simulink model "can_decoder"  (R2026a)
settings: configuration reference "AMCBLDC_Configuration" (kept outside this file)
undefined symbols (not defined in the file): CAN_ID_AMC, CAN_VOLT_REF_GAIN, CAN_VOLT_REF_SHIFT
settings Model: DataDictionary=amcbldc.sldd  Creator=upattacini  LastModifiedBy=rpumpo
settings ConfigSetRef: SourceName=AMCBLDC_Configuration

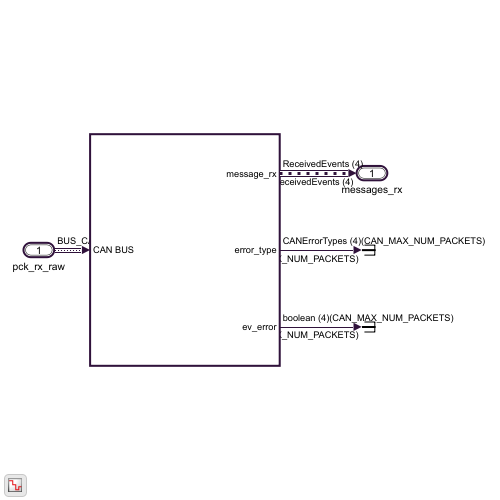
[thumbnail: Simulink's stored preview of the top-level diagram]
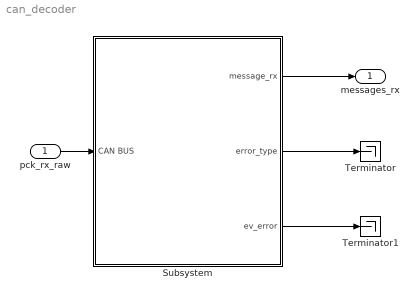
== system can_decoder ==
  pck_rx_raw : Inport  OutDataTypeStr=Bus: BUS_CAN_MULTIPLE  BusOutputAsStruct=on
  Subsystem : Subsystem
  Terminator : Terminator
  Terminator1 : Terminator
  messages_rx : Outport  OutDataTypeStr=Bus: ReceivedEvents  BusOutputAsStruct=on
  wires:
  pck_rx_raw/1 -> Subsystem/1(CAN BUS)
  Subsystem/1(message_rx) -> messages_rx/1
  Subsystem/2(error_type) -> Terminator/1
  Subsystem/3(ev_error) -> Terminator1/1

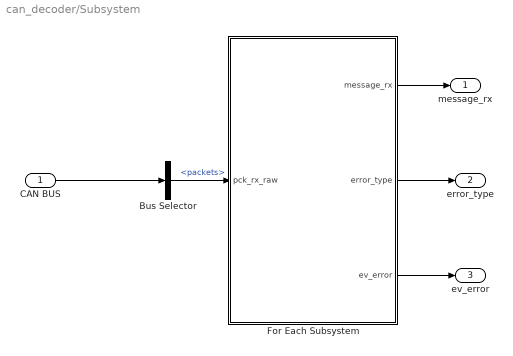
== system can_decoder/Subsystem ==
  CAN BUS : Inport
  Bus Selector : BusSelector  OutputSignals=packets
  For Each Subsystem : Subsystem  TreatAsAtomicUnit=on
  message_rx : Outport  PortDimensions=4
  error_type : Outport  Port=2
  ev_error : Outport  Port=3
  wires:
  Bus Selector/1 -> For Each Subsystem/1(pck_rx_raw)  "<packets>"
  CAN BUS/1 -> Bus Selector/1
  For Each Subsystem/3(ev_error) -> ev_error/1
  For Each Subsystem/1(message_rx) -> message_rx/1
  For Each Subsystem/2(error_type) -> error_type/1

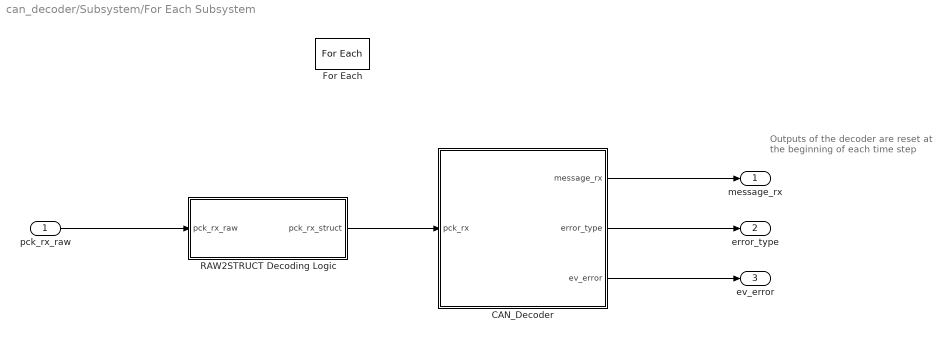
== system can_decoder/Subsystem/For Each Subsystem ==
  note: Outputs of the decoder are reset at
      | the beginning of each time step
  pck_rx_raw : Inport  Partition=on  PartitionDimension=1  PartitionWidth=1  PartitionOffset=0
  CAN_Decoder : Subsystem  TreatAsAtomicUnit=on
  For Each : ForEach  DisableCoverage=on  SpecifiedNumIters=MAX_EVENTS_PER_TICK
  RAW2STRUCT Decoding Logic : MATLAB Function  TreatAsAtomicUnit=on
  message_rx : Outport  OutDataTypeStr=Bus: ReceivedEvents  ConcatenationDimension=1
  error_type : Outport  Port=2  ConcatenationDimension=1
  ev_error : Outport  Port=3  ConcatenationDimension=1
  wires:
  CAN_Decoder/3(ev_error) -> ev_error/1
  RAW2STRUCT Decoding Logic/1(pck_rx_struct) -> CAN_Decoder/1(pck_rx)
  CAN_Decoder/1(message_rx) -> message_rx/1
  pck_rx_raw/1 -> RAW2STRUCT Decoding Logic/1(pck_rx_raw)
  CAN_Decoder/2(error_type) -> error_type/1

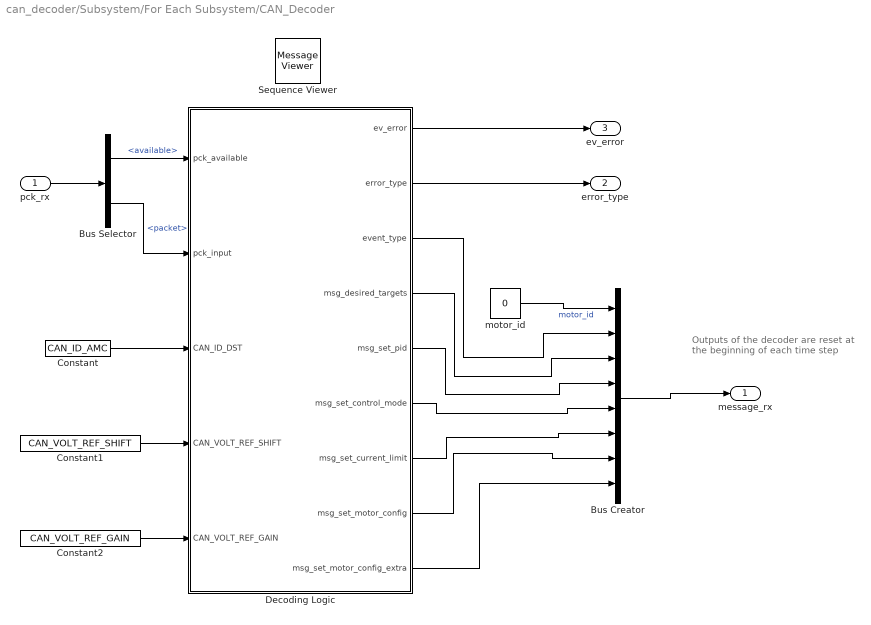
== system can_decoder/Subsystem/For Each Subsystem/CAN_Decoder ==
  note: Outputs of the decoder are reset at
      | the beginning of each time step
  pck_rx : Inport  OutDataTypeStr=Bus: BUS_CAN_RX
  Bus Creator : BusCreator  Inputs=8  OutDataTypeStr=Bus: ReceivedEvents  NonVirtualBus=on
      settings: InheritFromInputs=off
  Bus Selector : BusSelector  OutputSignals=available,packet
  Constant : Constant  Value=CAN_ID_AMC  OutDataTypeStr=uint8
  Constant1 : Constant  Value=CAN_VOLT_REF_SHIFT  OutDataTypeStr=uint8
  Constant2 : Constant  Value=CAN_VOLT_REF_GAIN  OutDataTypeStr=single
  Decoding Logic : Stateflow chart  TreatAsAtomicUnit=on
      settings: PortSchema="{\"entries\":[{\"content\":{\"sides\":[{\"content\":{\"connectorIds\":[\"In1\",\"In2\",\"In3\",\"In4\",\"In5\"]},\"type\":\"ConnectorPlacement.EquallySpacedRectSide\",\"uuid\":\"bb5ffdcb-390f-4d7b-9f99-b75bae8a05ad\"},{\"content\":{\"connectorIds\":[\"Out9\",\"Out6\",\"Out7\",\"Out3\",\"Out4\",\"Out1\",\"Out2\",\"Out5\",\"Out8\"],\"side\":\"RIGHT\"},\"type\":\"ConnectorPlacement.EquallySpacedRectSide\",\"uuid\":\"3ba90815-a3e4-4cd4-b64a-5c95e1f5d631\"},{\"content\":{\"side\":\"TOP\"},\"type\":\"ConnectorPlacement.EquallySpacedRectSide\",\"uuid\":\"c9c9b262-1031-4ca9-8b93-619604387376\"}]},\"type\":\"ConnectorPlacement.EquallySpacedConnector\",\"uuid\":\"025015ea-955c-40a8-a93e-b34368e10f0a\"}],\"packageUris\":[\"http://schema.mathworks.com/mf0/Connector/R2020b\"],\"version\":\"1.0\"}"
  Sequence Viewer : MessageViewer
  motor_id : Constant  Value=0  OutDataTypeStr=uint8
  message_rx : Outport  OutDataTypeStr=Bus: ReceivedEvents
  error_type : Outport  Port=2
  ev_error : Outport  Port=3
  wires:
  Constant/1 -> Decoding Logic/3(CAN_ID_DST)
  pck_rx/1 -> Bus Selector/1
  Bus Selector/1 -> Decoding Logic/1(pck_available)  "<available>"
  Bus Selector/2 -> Decoding Logic/2(pck_input)  "<packet>"
  Constant1/1 -> Decoding Logic/4(CAN_VOLT_REF_SHIFT)
  Constant2/1 -> Decoding Logic/5(CAN_VOLT_REF_GAIN)
  Decoding Logic/9(ev_error) -> ev_error/1
  Decoding Logic/6(error_type) -> error_type/1
  Bus Creator/1 -> message_rx/1
  Decoding Logic/7(event_type) -> Bus Creator/2
  Decoding Logic/3(msg_desired_targets) -> Bus Creator/3
  Decoding Logic/4(msg_set_pid) -> Bus Creator/4
  Decoding Logic/1(msg_set_control_mode) -> Bus Creator/5
  Decoding Logic/2(msg_set_current_limit) -> Bus Creator/6
  Decoding Logic/5(msg_set_motor_config) -> Bus Creator/7
  motor_id/1 -> Bus Creator/1  "motor_id"
  Decoding Logic/8(msg_set_motor_config_extra) -> Bus Creator/8

== matlab function can_decoder/Subsystem/For Each Subsystem/RAW2STRUCT Decoding Logic ==
  data: pck_rx_raw input Bus: BUS_CAN; pck_rx_struct output Bus: BUS_CAN_RX
function pck_rx_struct = raw2struct(pck_rx_raw)

pck_rx_struct.available = pck_rx_raw.available;

% ID
pck_rx_struct.packet.ID.CLS = CANClassTypes(bitshift(bitand(pck_rx_raw.packet.ID, 0x0700), -8));
pck_rx_struct.packet.ID.SRC = uint8(bitshift(bitand(pck_rx_raw.packet.ID, 0x0f0), -4));
pck_rx_struct.packet.ID.DST_TYP = uint8(bitand(pck_rx_raw.packet.ID, 0x00f));

% PAYLOAD
pck_rx_struct.packet.PAYLOAD.LEN = max([0, min([8, pck_rx_raw.length])]);
pck_rx_struct.packet.PAYLOAD.CMD.M = (bitand(pck_rx_raw.packet.PAYLOAD(1), 0x80) ~= 0);
pck_rx_struct.packet.PAYLOAD.CMD.OPC = bitand(pck_rx_raw.packet.PAYLOAD(1), 0x7f);
% We get both the polling and the streaming packtes covered
pck_rx_struct.packet.PAYLOAD.ARG = pck_rx_raw.packet.PAYLOAD;

== stateflow chart can_decoder/Subsystem/For Each Subsystem/CAN_Decoder/Decoding Logic ==
  settings: initializeOutput=1  description=This state chart is responsible for decoding incoming CAN packets.
  state ErrorHandler [parallel]
    settings: executionOrder=2
    state Home
      entry:
      cmd_processed = 0;
      exit:
      ev_async = false;
    state Event_Error
      entry:
      ev_async = true;
    (default) -> ErrorHandler.Home
    (junction 111) -> ErrorHandler.Home [order 2] : {error_type = CANErrorTypes.No_Error;}
    (junction 111) -> ErrorHandler.Home [order 1] : [cmd_processed > 1]
        | {error_type = CANErrorTypes.Packet_MultiFunctionsDetected;
        | send(ev_error);}
    ErrorHandler.Home -> ErrorHandler.Home [order 4] : [ev_async]
    (junction 109) -> ErrorHandler.Home [order 1] : [pck_available && (cmd_processed == 0)]
        | {error_type = CANErrorTypes.Packet_Unrecognized;
        | send(ev_error);}
    Event_Error -> ErrorHandler.Home
    ErrorHandler.Home -> (junction 109) [order 5]
    ErrorHandler.Home -> Event_Error [order 1] : ev_error_pck_not4us
        | {error_type = CANErrorTypes.Packet_Not4Us;
        | send(ev_error);}
    ErrorHandler.Home -> Event_Error [order 2] : ev_error_pck_malformed
        | {error_type = CANErrorTypes.Packet_Malformed;
        | send(ev_error);}
    ErrorHandler.Home -> Event_Error [order 3] : ev_error_mode_unrecognized
        | {error_type = CANErrorTypes.Mode_Unrecognized;
        | send(ev_error);}
    (junction 109) -> (junction 111) [order 2]
  state CANParser [parallel]
    settings: executionOrder=1
    state Home
    state SetCommand [function]
      state r = isPayloadValid(expected_size) [function]
        (default) -> (junction 402) : {r = true;}
        (junction 402) -> (junction 503) [order 1] : [pck_input.ID.DST_TYP != CAN_ID_DST]{send(ev_error_pck_not4us, ErrorHandler); r = false;}
        (junction 402) -> (junction 505) [order 2] : [pck_input.PAYLOAD.LEN < 1]{send(ev_error_pck_malformed, ErrorHandler); r = false;}
        (junction 402) -> (junction 507) [order 3] : [pck_input.PAYLOAD.LEN <  expected_size]
            | {send(ev_error_pck_malformed, ErrorHandler);; r = false;}
      state SetControlMode [function]
        (default) -> (junction 510)
        (junction 510) -> (junction 339) [order 2] : {mc_mode =  pck_input.PAYLOAD.ARG[1];}
        (junction 339) -> (junction 406) [order 2] : {% msg_set_control_mode.motor = pck_input.PAYLOAD.CMD.M;
            | msg_set_control_mode = convertMode(mc_mode);
            | cmd_processed++;
            | event_type = EventTypes.SetControlMode;}
        (junction 339) -> (junction 408) [order 1] : [!is_controlmode_recognized(mc_mode)]
            | {send(ev_error_mode_unrecognized, ErrorHandler);}
        (junction 510) -> (junction 523) [order 1] : [!isPayloadValid(2)]
      state SetCurrentLimits [function]
        (default) -> (junction 381)
        (junction 381) -> (junction 527) [order 1] : [!isPayloadValid(8)]
        (junction 381) -> (junction 382) [order 2] : {% msg_set_current_limit.motor = pck_input.PAYLOAD.CMD.M;
            | msg_set_current_limit.nominal = single(0.001)*single(merge_2bytes_signed(pck_input.PAYLOAD.ARG[2], pck_input.PAYLOAD.ARG[3]));
            | msg_set_current_limit.peak = single(0.001)*single(merge_2bytes_unsigned(pck_input.PAYLOAD.ARG[4], pck_input.PAYLOAD.ARG[5]));
            | msg_set_current_limit.overload = single(0.001)*single(merge_2bytes_unsigned(pck_input.PAYLOAD.ARG[6], pck_input.PAYLOAD.ARG[7]));
            | cmd_processed++;
            | event_type = EventTypes.SetLimit;}
      state SetMotorConfig [function]
        (default) -> (junction 397)
        (junction 397) -> (junction 530) [order 1] : [!isPayloadValid(8)]
        (junction 397) -> (junction 398) [order 2] : {msg_set_motor_config.has_quadrature_encoder = boolean(pck_input.PAYLOAD.ARG[1] & 0x01);
            | msg_set_motor_config.has_hall_sens = boolean(pck_input.PAYLOAD.ARG[1] & 0x02);
            | msg_set_motor_config.has_temperature_sens = boolean(pck_input.PAYLOAD.ARG[1] & 0x04);
            | msg_set_motor_config.use_index = boolean(pck_input.PAYLOAD.ARG[1] & 0x08);
            | msg_set_motor_config.has_speed_quadrature_encoder = boolean(pck_input.PAYLOAD.ARG[1] & 0x10);
            | msg_set_motor_config.enable_verbosity = boolean(pck_input.PAYLOAD.ARG[1] & 0x20);
            | msg_set_motor_config.rotor_encoder_resolution = merge_2bytes_signed(pck_input.PAYLOAD.ARG[2], pck_input.PAYLOAD.ARG[3]);
            | msg_set_motor_config.rotor_index_offset = merge_2bytes_signed(pck_input.PAYLOAD.ARG[4], pck_input.PAYLOAD.ARG[5]);
            | msg_set_motor_config.pole_pairs = pck_input.PAYLOAD.ARG[6] / 2;
            | msg_set_motor_config.encoder_tolerance = pck_input.PAYLOAD.ARG[7];
            | cmd_processed++;
            | event_type = EventTypes.SetMotorConfig;}
      state SetCurrentPID [function]
        (default) -> (junction 386)
        (junction 386) -> (junction 387) [order 2] : {%msg_set_pid.motor = pck_input.PAYLOAD.CMD.M;
            | msg_set_pid.shift_factor = pck_input.PAYLOAD.ARG[7];
            | c = single(0x01 << (15 - msg_set_pid.shift_factor)) / single(32768);
            | msg_set_pid.P = c * single(merge_2bytes_signed(pck_input.PAYLOAD.ARG[1], pck_input.PAYLOAD.ARG[2]));
            | msg_set_pid.I = c * single(merge_2bytes_signed(pck_input.PAYLOAD.ARG[3], pck_input.PAYLOAD.ARG[4]));
            | msg_set_pid.D = c * single(merge_2bytes_signed(pck_input.PAYLOAD.ARG[5], pck_input.PAYLOAD.ARG[6]));
            | msg_set_pid.type = ControlModes.Current;
            | event_type = EventTypes.SetPid;
            | cmd_processed++;}
        (junction 386) -> (junction 532) [order 1] : [!isPayloadValid(8)]
      state SetVelocityPID [function]
        (default) -> (junction 391)
        (junction 391) -> (junction 392) [order 2] : {msg_set_pid.shift_factor = pck_input.PAYLOAD.ARG[7];
            | c = single(0x01 << (15 - msg_set_pid.shift_factor)) / single(32768);
            | msg_set_pid.P = c * single(merge_2bytes_signed(pck_input.PAYLOAD.ARG[1], pck_input.PAYLOAD.ARG[2]));
            | msg_set_pid.I = c * single(merge_2bytes_signed(pck_input.PAYLOAD.ARG[3], pck_input.PAYLOAD.ARG[4]));
            | msg_set_pid.D = c * single(merge_2bytes_signed(pck_input.PAYLOAD.ARG[5], pck_input.PAYLOAD.ARG[6]));
            | msg_set_pid.P *= single(0.001);
            | msg_set_pid.I *= single(0.001);
            | msg_set_pid.D *= single(0.001);
            | msg_set_pid.type = ControlModes.Velocity;
            | event_type = EventTypes.SetPid;
            | cmd_processed++;}
        (junction 391) -> (junction 534) [order 1] : [!isPayloadValid(8)]
      state SetPositionPID [function]
        (default) -> (junction 826)
        (junction 826) -> (junction 827) [order 2] : {msg_set_pid.shift_factor = pck_input.PAYLOAD.ARG[7];
            | c = single(0x01 << (15 - msg_set_pid.shift_factor)) / single(32768);
            | msg_set_pid.P = c * single(merge_2bytes_signed(pck_input.PAYLOAD.ARG[1], pck_input.PAYLOAD.ARG[2]));
            | msg_set_pid.I = c * single(merge_2bytes_signed(pck_input.PAYLOAD.ARG[3], pck_input.PAYLOAD.ARG[4]));
            | msg_set_pid.D = c * single(merge_2bytes_signed(pck_input.PAYLOAD.ARG[5], pck_input.PAYLOAD.ARG[6]));
            | msg_set_pid.type = ControlModes.Position;
            | event_type = EventTypes.SetPid;
            | cmd_processed++;}
        (junction 826) -> (junction 825) [order 1] : [!isPayloadValid(8)]
      state SetMotorParameter [function]
        (default) -> (junction 747)
        (junction 747) -> (junction 731) [order 2] : {p = pck_input.PAYLOAD.ARG[1];}
        (junction 731) -> (junction 722) [order 1] : [p == MCMotorParamsSet.Kbemf]
        (junction 722) -> (junction 715) : {msg_set_motor_config_extra.value = ...
            | merge_4bytes_single(pck_input.PAYLOAD.ARG);}
        (junction 747) -> (junction 809) [order 1] : [!isPayloadValid(8)]
        (junction 731) -> (junction 718) [order 2]
        (junction 715) -> (junction 714)
        (junction 718) -> (junction 719) [order 1] : [p == MCMotorParamsSet.hall]
        (junction 719) -> (junction 714) : {msg_set_motor_config_extra.value = ...
            | unpack_hall_config(pck_input.PAYLOAD.ARG);}
        (junction 718) -> (junction 717) [order 2]
        (junction 714) -> (junction 738)
        (junction 717) -> (junction 723) [order 1] : [p == MCMotorParamsSet.elect_vmax]
        (junction 723) -> (junction 738) : {msg_set_motor_config_extra.value = ...
            | merge_4bytes_single(pck_input.PAYLOAD.ARG);}
        (junction 717) -> (junction 740) [order 2]
        (junction 738) -> (junction 739)
        (junction 739) -> (junction 740) : {msg_set_motor_config_extra.key = p;}
        (junction 740) -> (junction 742) : {event_type = EventTypes.SetMotorParam;}
      state Set [function]
        (default) -> (junction 877)
        (junction 877) -> (junction 878) : [(pck_input.PAYLOAD.LEN == 8) && (CAN_ID_DST <= 4)]
            | {
            |  [msg_desired_targets.position,msg_desired_targets.velocity] = decode_pos_vel(pck_input.PAYLOAD.ARG);
            | cmd_processed++;
            | event_type = EventTypes.SetTarget;}
      (default) -> (junction 310)
      (junction 310) -> (junction 312) [order 1] : [pck_input.PAYLOAD.CMD.OPC == MCOPC.Set_Control_Mode]
          | {SetControlMode();}
      (junction 310) -> (junction 314) [order 2]
      (junction 312) -> (junction 316)
      (junction 314) -> (junction 316) [order 1] : [pck_input.PAYLOAD.CMD.OPC == MCOPC.Set_Current_Limit]
          | {SetCurrentLimits();}
      (junction 314) -> (junction 318) [order 2]
      (junction 316) -> (junction 321)
      (junction 318) -> (junction 321) [order 1] : [pck_input.PAYLOAD.CMD.OPC == MCOPC.Set_Motor_Config]
          | {SetMotorConfig();}
      (junction 318) -> (junction 324) [order 2]
      (junction 321) -> (junction 322)
      (junction 324) -> (junction 322) [order 1] : [pck_input.PAYLOAD.CMD.OPC == MCOPC.Set_Current_PID]
          | {SetCurrentPID();}
      (junction 324) -> (junction 328) [order 2]
      (junction 322) -> (junction 326)
      (junction 328) -> (junction 326) [order 1] : [pck_input.PAYLOAD.CMD.OPC == MCOPC.Set_Velocity_PID]
          | {SetVelocityPID();}
      (junction 326) -> (junction 819)
      (junction 328) -> (junction 821) [order 2]
      (junction 821) -> (junction 819) [order 1] : [pck_input.PAYLOAD.CMD.OPC == MCOPC.Set_Position_PID]
          | {SetPositionPID();}
      (junction 821) -> (junction 614) [order 2]
      (junction 819) -> (junction 618)
      (junction 614) -> (junction 618) [order 1] : [pck_input.PAYLOAD.CMD.OPC == MCOPC.Set_Parameter]
          | {SetMotorParameter();}
      (junction 618) -> (junction 576)
      (junction 614) -> (junction 334) [order 2]
      (junction 334) -> (junction 576) [order 1] : [pck_input.PAYLOAD.CMD.OPC == MCOPC.Set]
          | {Set();}
      (junction 334) -> (junction 831) [order 2]
      (junction 576) -> (junction 834)
      (junction 834) -> (junction 831)
      (junction 831) -> (junction 579)
    state SetStreaming [function]
      state SetTargets [function]
        (default) -> (junction 372)
        (junction 372) -> (junction 373) : [(pck_input.PAYLOAD.LEN == 8) && (CAN_ID_DST <= 4)]
            | {idx = 2*(CAN_ID_DST-1);
            | tmp_merged = merge_2bytes_signed(pck_input.PAYLOAD.ARG[idx], pck_input.PAYLOAD.ARG[idx+1]);
            | msg_desired_targets.current = single(0.001) * single(tmp_merged);
            | msg_desired_targets.voltage = single(tmp_merged >> CAN_VOLT_REF_SHIFT) / CAN_VOLT_REF_GAIN;
            | msg_desired_targets.velocity = single(1000) * single(tmp_merged) * CAN_ANGLE_ICUB2DEG;
            | cmd_processed++;
            | event_type = EventTypes.SetTarget;}
      (default) -> (junction 344)
      (junction 344) -> (junction 345) : [ (MCStreaming(pck_input.ID.DST_TYP) == MCStreaming.Desired_Targets)]
          | {SetTargets();}
    (default) -> CANParser.Home
    CANParser.Home -> (junction 535) : [pck_available]
    (junction 535) -> (junction 303) [order 1] : [(pck_input.ID.CLS == CANClassTypes.Motor_Control_Command)]
        | {SetCommand();}
    (junction 535) -> CANParser.Home [order 3]
    (junction 535) -> (junction 303) [order 2] : [(pck_input.ID.CLS == CANClassTypes.Motor_Control_Streaming)]
        | {SetStreaming();}
    (junction 303) -> CANParser.Home
  data: ev_async local boolean =false; expected_size function_input uint8; r function_output boolean; MCMode function_input Enum: MCControlModes; mode function_output Enum: ControlModes; mode function_input int32; ok function_output boolean; d function_input uint8 size=8; sw function_output single size=[2, 1]; hall_data function_output single size=[2, 1]; d function_input uint8 size=8; payload function_input uint8 size=[1,8]; target_pos function_output single; target_vel function_output single; hex function_input uint16; decimal_value function_output single; bl function_input uint16; bh function_input uint16; uw function_output uint16; bl function_input uint16; bh function_input uint16; sw function_output int16; pck_available input boolean; pck_input input Bus: BUS_CAN_PACKET_RX; CAN_ID_DST input uint8; msg_set_control_mode output Enum: ControlModes; msg_set_current_limit output Bus: SupervisorInputLimits; msg_desired_targets output Bus: Targets; msg_set_pid output Bus: PID; msg_set_motor_config output Bus: MotorConfigurationExternal; error_type output Enum: CANErrorTypes size=1 =CANErrorTypes.No_Error; cmd_processed local uint16 size=1 =0; CAN_VOLT_REF_SHIFT input uint8; CAN_VOLT_REF_GAIN input single; CAN_ANGLE_ICUB2DEG parameter; event_type output Enum: EventTypes =EventTypes.None; c local double; tmp_merged local double; idx local double; mc_mode local double; p local uint8; msg_set_motor_config_extra output Bus: MotorConfigurationExtSet
  data CAN_ID_DST settings: description=The ID of the receiver.
  data msg_set_control_mode settings: description=Contains the data to set the required control mode.
  data msg_set_current_limit settings: description=Contains the data to set the required current limit.
  data msg_desired_targets settings: description=Contains the data to set the required current limit.
  data msg_set_pid settings: description=Contains the data to set the required current limit.
  data msg_set_motor_config settings: description=Contains the data to set the required current limit.
  events: ev_error_mode_unrecognized local FUNCTION_CALL_EVENT; ev_error output EITHER_EDGE_EVENT; ev_error_pck_malformed local FUNCTION_CALL_EVENT; ev_error_pck_not4us local FUNCTION_CALL_EVENT
  function mode = convertMode(MCMode):
    | function mode = convertMode(MCMode)
    | 
    |     if MCMode == MCControlModes.Idle
    |         mode = ControlModes.Idle;
    |     elseif MCMode == MCControlModes.Current
    |         mode = ControlModes.Current;
    |     elseif MCMode == MCControlModes.SpeedVoltage
    |         mode = ControlModes.Velocity;
    |     elseif MCMode == MCControlModes.OpenLoop
    |         mode = ControlModes.Voltage;
    |     elseif MCMode == MCControlModes.Position
    |         mode = ControlModes.Position;
    |     else
    |         mode = ControlModes.Idle;
    |     end
    | 
    | end
  function ok = is_controlmode_recognized(mode):
    | function ok = is_controlmode_recognized(mode) 
    | 
    | ok = true;
    | if (mode ~= MCControlModes.Idle)         && ...
    |    (mode ~= MCControlModes.OpenLoop)     && ...
    |    (mode ~= MCControlModes.SpeedVoltage) && ...
    |    (mode ~= MCControlModes.Current)      && ...
    |    (mode ~= MCControlModes.Position)
    |     ok = false;
    | end
  function sw = merge_4bytes_single(d):
    | function sw = merge_4bytes_single(d)
    | par = d(3:6);
    | sw = single([.0; .0]);
    | sw(1) = single(typecast(par(1:1:end), 'single'));
  function hall_data = unpack_hall_config(d):
    | function hall_data = unpack_hall_config(d)
    | 
    | hall_data = single([0.0; 0.0]);
    | 
    | hall_data(1) = single(typecast([d(3), d(4)], "int16"));
    | 
    | % get the nibble from payload byte 4
    | % assuming the nibble we want is the most significant
    | % part of the byte
    | % hall_data(2) = single(bitshift(d(5), -4));
    | hall_data(2) = single(d(5));
  function [target_pos,target_vel] = decode_pos_vel(payload):
    | function  [target_pos,target_vel] = decode_pos_vel(payload)
    | bytes_pos = payload(3:6); 
    | target_pos = typecast(bytes_pos, 'single');
    | 
    | bytes_vel = payload(7:8);
    | 
    | 
    | hex = typecast(bytes_vel, 'uint16'); 
    | target_vel = hexHalfToSingle(hex);
  function decimal_value = hexHalfToSingle(hex):
    | function decimal_value = hexHalfToSingle(hex)
    |     h = uint16(hex);
    |     
    |     % If it's zero, return zero immediately
    |     if h == 0
    |         decimal_value = single(0);
    |         return;
    |     end
    |     
    |     % Ensure h is uint16 for correct use with bitwise operations
    |     h = uint16(h);
    |     
    |     % Constants for the Half-Float format (1-5-10 bit)
    |     SIGN_MASK = uint16(0x8000); % 1000 0000 0000 0000
    |     EXP_MASK  = uint16(0x7C00); % 0111 1100 0000 0000
    |     MAN_MASK  = uint16(0x03FF); % 0000 0011 1111 1111
    |     
    |     % Exponent Bias (difference between float32 bias 127 and float16 bias 15)
    |     EXP_BIAS_DIFF = uint32(127 - 15); 
    |     
    |     % --- Half-Float Field Extraction ---
    |     
    |     % 1. Sign (shifted to position 31 for float32)
    |     sign = bitshift(uint32(bitand(h, SIGN_MASK)), 16);
    |     
    |     % 2. Exponent (raw)
    |     exp_h = bitshift(bitand(h, EXP_MASK), -10);
    |     
    |     % 3. Mantissa (raw)
    |     man_h = bitand(h, MAN_MASK);
    |     
    |     % --- Conversion to Float32 (uint32 representation) ---
    |     if exp_h == 0 % Denormals and Zero (zero already handled above)
    |         
    |         % Denormals are complex; for simplicity, we treat them basically. 
    |         % A complete implementation would require floating-point calculations.
    |         
    |         % In a complete implementation they should be handled differently,
    |         % but for normal values like 6DDC this block is not executed.
    |         u_f = bitshift(uint32(man_h), uint32(23-10));
    |         
    |     elseif exp_h == 31 % Infinity and NaN (not handled for simplicity, pattern is returned)
    |         
    |         u_f = bitor(sign, bitor(bitshift(uint32(31), 23), bitshift(uint32(man_h), 13)));
    |     else % Normal values
    |         
    |         % Re-calculate the exponent: add the Bias difference
    |         exp_f = uint32(exp_h) + EXP_BIAS_DIFF;
    |         
    |         % Shift the exponent to the float32 position (23)
    |         exp_f_shifted = bitshift(exp_f, 23);
    |         
    |         % Shift the mantissa by 13 positions (10 bit -> 23 bit)
    |         man_f_shifted = bitshift(uint32(man_h), 13);
    |         
    |         % Combine the three fields into the float32 binary pattern (uint32)
    |         u_f = bitor(sign, bitor(exp_f_shifted, man_f_shifted));
    |     end
    |     
    |     decimal_value = typecast(u_f, 'single');
    | end
  function uw = merge_2bytes_unsigned(bl, bh):
    | function uw = merge_2bytes_unsigned(bl, bh)
    | 
    | uw = bitor(bitshift(bh, 8), bl);
  function sw = merge_2bytes_signed(bl, bh):
    | function sw = merge_2bytes_signed(bl, bh)
    | 
    | uw = bitor(bitshift(bh, 8), bl);
    | sw = typecast(uw, 'int16');
